simulink model "rocket_sim"  (R2023a)
settings: Solver=VariableStepAuto  StartTime=0.0  StopTime=480  RelTol=1e-3
undefined symbols (not defined in the file or in its folder): Earth, WGS84
libraries: simulink x55, slpidlib x10, aerolibconvert2 x7, matrix_library x4, aerolibasang x3, aerolibtransform2 x2, aerolibatmos2 x2, shared6dof x1, sharedtransform x1
(part 2 of 3)

== system rocket_sim/制导模块/Subsystem ==
  Clock2 : Clock
  Constant10 : Constant  Value=549000
  Constant11 : Constant  Value=150
  Constant12 : Constant  Value=486000
  Constant13 : Constant  Value=405000
  Gain2 : Gain  Gain=2700
  Gain3 : Gain  Gain=900
  Sum4 : Sum  Inputs=|+-
  Sum5 : Sum  Inputs=|+-
  Sum6 : Sum  Inputs=|++
  Switch4 : Switch  Criteria=u2 > Threshold  Threshold=150  SaturateOnIntegerOverflow=off  InputSameDT=off
  Switch5 : Switch  Criteria=u2 > Threshold  Threshold=240  SaturateOnIntegerOverflow=off  InputSameDT=off
  Out1 : Outport
  wires:
  Sum6/1 -> Switch5/3
  Gain2/1 -> Switch4/3
  Clock2/1 -> Switch5/2, Sum5/1, Switch4/2, Gain2/1
  Sum5/1 -> Gain3/1
  Constant10/1 -> Sum4/1
  Gain3/1 -> Sum6/1
  Constant12/1 -> Switch5/1
  Switch5/1 -> Switch4/1
  Sum4/1 -> Out1/1
  Constant13/1 -> Sum6/2
  Switch4/1 -> Sum4/2
  Constant11/1 -> Sum5/2

== system rocket_sim/制导模块/Subsystem1 ==
  Clock1 : Clock
  Constant : Constant  Value=[7000000;0;0]
  Constant3 : Constant  Value=[0;0;0]
  Constant8 : Constant  Value=[2000000;0;0]
  Constant9 : Constant  Value=[800000;0;0]
  Switch1 : Switch  Threshold=315  SaturateOnIntegerOverflow=off  InputSameDT=off
  Switch2 : Switch  Threshold=150  SaturateOnIntegerOverflow=off  InputSameDT=off
  Switch3 : Switch  Threshold=240  SaturateOnIntegerOverflow=off  InputSameDT=off
  Out1 : Outport
  wires:
  Clock1/1 -> Switch1/2, Switch3/2, Switch2/2
  Switch1/1 -> Switch3/1
  Constant3/1 -> Switch1/3
  Constant8/1 -> Switch3/3
  Constant9/1 -> Switch1/1
  Constant/1 -> Switch2/3
  Switch3/1 -> Switch2/1
  Switch2/1 -> Out1/1

== system rocket_sim/动力系统模块/喷管 ==
  dm : Inport
  P0 : Inport  Port=2
  Pi : Inport  Port=3
  Fwg : Inport  Port=4
  Th : Inport  Port=5
  F01 : Subsystem
  S71 : Scope
  喷管 : MATLAB Function  TreatAsAtomicUnit=on
  F : Outport
  ve : Outport  Port=2
  wires:
  dm/1 -> 喷管/1(dm)
  喷管/1(F) -> F/1
  Pi/1 -> 喷管/3(Pi)
  P0/1 -> 喷管/2(P0)
  喷管/2(ve) -> ve/1
  Fwg/1 -> F01/1(Fwg)
  Th/1 -> F01/2(Th)
  F01/1(Fwg1) -> S71/1, 喷管/4(Fwg1)

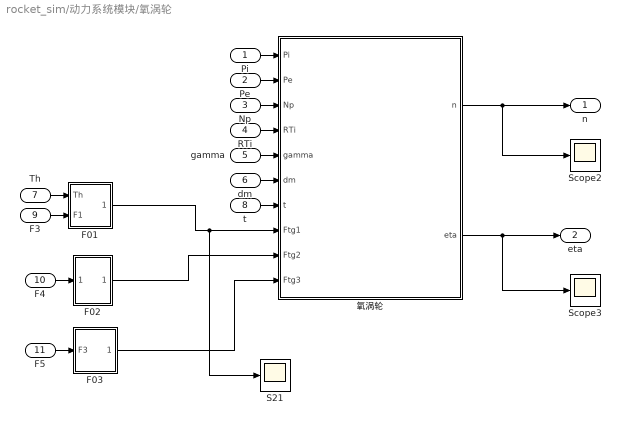
== system rocket_sim/动力系统模块/氧涡轮 ==
  Pi : Inport
  Pe : Inport  Port=2
  Np : Inport  Port=3
  RTi : Inport  Port=4
  gamma : Inport  Port=5
  dm : Inport  Port=6
  Th : Inport  Port=7
  t : Inport  Port=8
  F3 : Inport  Port=9
  F4 : Inport  Port=10
  F5 : Inport  Port=11
  F01 : Subsystem
  F02 : Subsystem
  F03 : Subsystem
  S21 : Scope
  Scope2 : Scope
  Scope3 : Scope
  氧涡轮 : MATLAB Function  TreatAsAtomicUnit=on
  n : Outport
  eta : Outport  Port=2
  wires:
  Pi/1 -> 氧涡轮/1(Pi)
  F03/1(Ftg3) -> 氧涡轮/10(Ftg3)
  Pe/1 -> 氧涡轮/2(Pe)
  Np/1 -> 氧涡轮/3(Np)
  F02/1(Ftg2) -> 氧涡轮/9(Ftg2)
  Th/1 -> F01/1(Th)
  t/1 -> 氧涡轮/7(t)
  F01/1(Ftg1) -> S21/1, 氧涡轮/8(Ftg1)
  F3/1 -> F01/2(F1)
  F4/1 -> F02/1(F2)
  RTi/1 -> 氧涡轮/4(RTi)
  F5/1 -> F03/1(F3)
  氧涡轮/2(eta) -> Scope3/1, eta/1
  dm/1 -> 氧涡轮/6(dm)
  氧涡轮/1(n) -> Scope2/1, n/1
  gamma/1 -> 氧涡轮/5(gamma)

== system rocket_sim/动力系统模块/液氧主阀 ==
  Pi : Inport
  dmi : Inport  Port=2
  Th : Inport  Port=3
  Constant : Constant
  F01 : Subsystem
  MATLAB Function : MATLAB Function  TreatAsAtomicUnit=on
  Memory : Memory
  S151 : Scope
  Pe : Outport
  dmo : Outport  Port=2
  wires:
  dmi/1 -> MATLAB Function/2(dmi)
  Pi/1 -> MATLAB Function/1(Pi)
  MATLAB Function/1(Pe) -> Pe/1
  Th/1 -> F01/1(Th)
  Constant/1 -> F01/2(Fv)
  F01/1(Fv1) -> S151/1, MATLAB Function/3(Fv1)
  Memory/1 -> dmo/1
  MATLAB Function/2(dmo) -> Memory/1

== system rocket_sim/动力系统模块/液氧泵 ==
  Pi : Inport
  n : Inport  Port=2
  Th : Inport  Port=3
  F1 : Inport  Port=4
  dm : Inport  Port=5
  F01 : Subsystem
  Memory : Memory
  S11 : Scope
  液氧泵 : MATLAB Function  TreatAsAtomicUnit=on
  Pe : Outport
  Np : Outport  Port=2
  dm02 : Outport  Port=3
  wires:
  Pi/1 -> 液氧泵/1(Pi)
  n/1 -> 液氧泵/3(n)
  F01/1(F) -> S11/1, 液氧泵/4(Fp1)
  液氧泵/1(Pe) -> Pe/1
  [dm] -> 液氧泵/2(dm)
  液氧泵/2(Np) -> Memory/1
  Memory/1 -> Np/1
  F1/1 -> F01/2(F1)
  Th/1 -> F01/1(Th)
  dm/1 -> [dm]
  [dm] -> dm02/1

== system rocket_sim/动力系统模块/液氧管路 ==
  P_i : Inport
  dm_i : Inport  Port=2
  Th : Inport  Port=3
  Constant6 : Constant
  F : Constant
  F01 : Subsystem
  Gain : Gain  Gain=0.02
  Integrator2 : Integrator
  MATLAB Function : MATLAB Function  TreatAsAtomicUnit=on
  Memory : Memory
  S141 : Scope
  dm_o : Outport
  P_e : Outport  Port=2
  dm_s1 : Outport  Port=3
  wires:
  P_i/1 -> MATLAB Function/1(P_i)
  Constant6/1 -> MATLAB Function/5(Fl2)
  MATLAB Function/2(P_e) -> P_e/1
  Integrator2/1 -> MATLAB Function/3(m)
  dm_i/1 -> Integrator2/1, MATLAB Function/2(dm_i)
  F01/1(F) -> S141/1, MATLAB Function/4(Fl1)
  Th/1 -> F01/1(Th)
  Gain/1 -> dm_s1/1
  MATLAB Function/1(dm_o) -> Memory/1
  Memory/1 -> Gain/1, dm_o/1
  F/1 -> F01/2(F1)

== system rocket_sim/动力系统模块/液氧贮箱 ==
  Band-Limited White Noise1 : simulink/Sources/Band-Limited White Noise  Cov=[0.1]  Ts=1  seed=[23341]
  Constant9 : Constant  Value=0.45
  Integrator1 : Integrator
  Step : Step  Time=0  After=214.06  SampleTime=0
  Sum : Sum  Inputs=|++
  σ1 : Gain  Gain=1e-3
  Po : Outport
  dm : Outport  Port=2
  wires:
  Constant9/1 -> Po/1
  Integrator1/1 -> σ1/1
  Band-Limited White Noise1/1 -> Integrator1/1
  Step/1 -> Sum/1
  Sum/1 -> dm/1
  σ1/1 -> Sum/2

== system rocket_sim/动力系统模块/煤油主阀 ==
  Pi : Inport
  dmi : Inport  Port=2
  Th : Inport  Port=3
  Fv : Inport  Port=4
  F01 : Subsystem
  MATLAB Function : MATLAB Function  TreatAsAtomicUnit=on
  Memory : Memory
  S41 : Scope
  Pe : Outport
  dmo : Outport  Port=2
  wires:
  F01/1(Fv1) -> S41/1, MATLAB Function/3(Fv1)
  dmi/1 -> MATLAB Function/2(dmi)
  Fv/1 -> F01/2(Fv)
  Pi/1 -> MATLAB Function/1(Pi)
  MATLAB Function/1(Pe) -> Pe/1
  Th/1 -> F01/1(Th)
  Memory/1 -> dmo/1
  MATLAB Function/2(dmo) -> Memory/1

== system rocket_sim/动力系统模块/煤油泵 ==
  Pi : Inport
  n : Inport  Port=2
  Th : Inport  Port=3
  dm : Inport  Port=4
  Constant : Constant
  F01 : Subsystem
  Memory : Memory
  S161 : Scope
  煤油泵 : MATLAB Function  TreatAsAtomicUnit=on
  Pe : Outport
  Np : Outport  Port=2
  dm12 : Outport  Port=3
  wires:
  Pi/1 -> 煤油泵/1(Pi)
  n/1 -> 煤油泵/3(n)
  F01/1(F) -> S161/1, 煤油泵/4(Fp1)
  煤油泵/1(Pe) -> Pe/1
  [dm] -> 煤油泵/2(dm)
  煤油泵/2(Np) -> Memory/1
  Memory/1 -> Np/1
  Constant/1 -> F01/2(F1)
  Th/1 -> F01/1(Th)
  dm/1 -> [dm]
  [dm] -> dm12/1

== system rocket_sim/动力系统模块/煤油涡轮 ==
  Pi : Inport
  Pe : Inport  Port=2
  Np : Inport  Port=3
  RTi : Inport  Port=4
  gamma : Inport  Port=5
  dm : Inport  Port=6
  Th : Inport  Port=7
  t : Inport  Port=8
  Constant : Constant
  Constant1 : Constant
  Constant2 : Constant
  F01 : Subsystem
  F02 : Subsystem
  F03 : Subsystem
  S171 : Scope
  Scope2 : Scope
  Scope3 : Scope
  氧涡轮 : MATLAB Function  TreatAsAtomicUnit=on
  n : Outport
  eta : Outport  Port=2
  wires:
  Pi/1 -> 氧涡轮/1(Pi)
  F03/1(Ftg3) -> 氧涡轮/10(Ftg3)
  Pe/1 -> 氧涡轮/2(Pe)
  Np/1 -> 氧涡轮/3(Np)
  F02/1(Ftg2) -> 氧涡轮/9(Ftg2)
  Th/1 -> F01/1(Th)
  t/1 -> 氧涡轮/7(t)
  F01/1(Ftg1) -> S171/1, 氧涡轮/8(Ftg1)
  RTi/1 -> 氧涡轮/4(RTi)
  氧涡轮/2(eta) -> Scope3/1, eta/1
  dm/1 -> 氧涡轮/6(dm)
  氧涡轮/1(n) -> Scope2/1, n/1
  gamma/1 -> 氧涡轮/5(gamma)
  Constant/1 -> F01/2(F1)
  Constant1/1 -> F02/1(F2)
  Constant2/1 -> F03/1(F3)

== system rocket_sim/动力系统模块/煤油管路 ==
  P_i : Inport
  dm_i : Inport  Port=2
  Th : Inport  Port=3
  Fl1 : Inport  Port=4
  Constant6 : Constant
  F01 : Subsystem
  Gain : Gain  Gain=0.02
  Integrator2 : Integrator
  MATLAB Function : MATLAB Function  TreatAsAtomicUnit=on
  Memory : Memory
  S31 : Scope
  dm_o : Outport
  P_e : Outport  Port=2
  dm_s1 : Outport  Port=3
  wires:
  P_i/1 -> MATLAB Function/1(P_i)
  Constant6/1 -> MATLAB Function/5(Fl2)
  MATLAB Function/2(P_e) -> P_e/1
  Integrator2/1 -> MATLAB Function/3(m)
  dm_i/1 -> Integrator2/1, MATLAB Function/2(dm_i)
  F01/1(F) -> S31/1, MATLAB Function/4(Fl1)
  Th/1 -> F01/1(Th)
  Fl1/1 -> F01/2(F1)
  Gain/1 -> dm_s1/1
  MATLAB Function/1(dm_o) -> Memory/1
  Memory/1 -> Gain/1, dm_o/1

== system rocket_sim/动力系统模块/煤油贮箱 ==
  Band-Limited White Noise1 : simulink/Sources/Band-Limited White Noise  Cov=[0.1]  Ts=1  seed=[23341]
  Constant9 : Constant  Value=0.31
  Integrator1 : Integrator
  Step : Step  Time=0  After=95.39  SampleTime=0
  Sum : Sum  Inputs=|++
  σ1 : Gain  Gain=1e-3
  Po : Outport
  dm : Outport  Port=2
  wires:
  Constant9/1 -> Po/1
  Band-Limited White Noise1/1 -> Integrator1/1
  Integrator1/1 -> σ1/1
  Step/1 -> Sum/1
  σ1/1 -> Sum/2
  Sum/1 -> dm/1

== system rocket_sim/动力系统模块/燃气发生器 ==
  dmo : Inport
  dmf : Inport  Port=2
  dmg : Inport  Port=3
  Pe : Inport  Port=4
  Th : Inport  Port=5
  F5 : Inport  Port=6
  Constant : Constant
  F01 : Subsystem
  S51 : Scope
  Scope : Scope
  燃气发生器 : MATLAB Function  TreatAsAtomicUnit=on
  gamma : Outport
  RT : Outport  Port=2
  dme : Outport  Port=3
  P : Outport  Port=4
  wires:
  dmg/1 -> 燃气发生器/3(dmg)
  Pe/1 -> 燃气发生器/4(Pe)
  燃气发生器/4(P) -> P/1
  dmo/1 -> 燃气发生器/1(dmo)
  dmf/1 -> 燃气发生器/2(dmf)
  Constant/1 -> 燃气发生器/5(Fg1)
  燃气发生器/1(gamma) -> gamma/1
  燃气发生器/2(RT) -> RT/1
  燃气发生器/3(dme) -> dme/1
  Th/1 -> F01/1(Th)
  F5/1 -> F01/2(F5)
  F01/1(Fg2) -> S51/1, 燃气发生器/6(Fg2)

== system rocket_sim/动力系统模块/燃烧室 ==
  dmo : Inport
  dmf : Inport  Port=2
  dmg : Inport  Port=3
  Th : Inport  Port=4
  Fr : Inport  Port=5
  F01 : Subsystem
  S61 : Scope
  燃烧室 : MATLAB Function  TreatAsAtomicUnit=on
  Pe : Outport
  dm : Outport  Port=2
  wires:
  dmg/1 -> 燃烧室/3(dmg)
  dmf/1 -> 燃烧室/2(dmf)
  燃烧室/1(Pe) -> Pe/1
  燃烧室/2(dm) -> dm/1
  dmo/1 -> 燃烧室/1(dmo)
  F01/1(Fr1) -> S61/1, 燃烧室/4(Fr1)
  Th/1 -> F01/1(Th)
  Fr/1 -> F01/2(Fr)

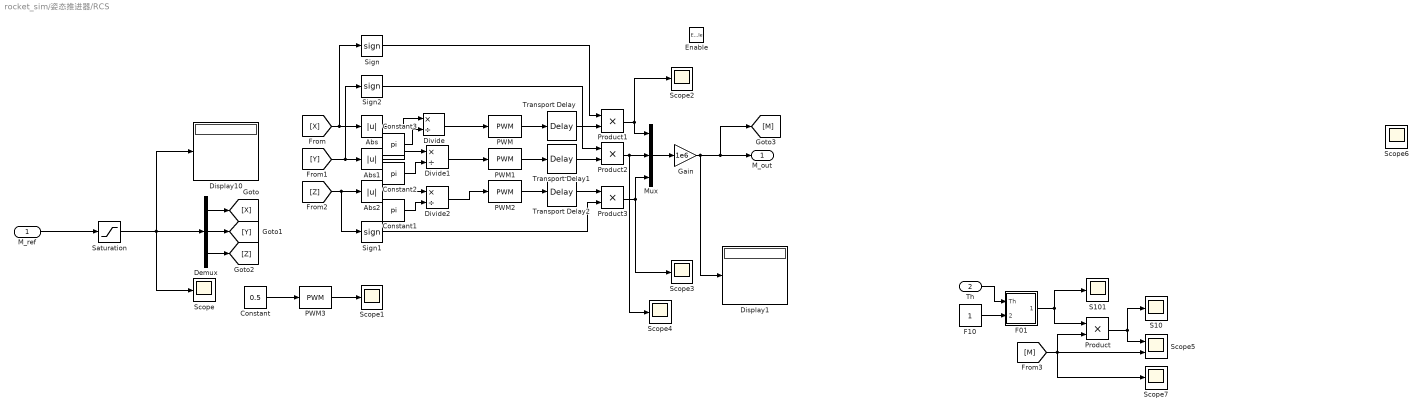
== system rocket_sim/姿态推进器/RCS ==
  M_ref : Inport
  Th : Inport  Port=2
  Enable : EnablePort
  Abs : Abs  SaturateOnIntegerOverflow=off
  Abs1 : Abs  SaturateOnIntegerOverflow=off
  Abs2 : Abs  SaturateOnIntegerOverflow=off
  Constant : Constant  Value=0.5
  Constant1 : Constant  Value=pi
  Constant2 : Constant  Value=pi
  Constant3 : Constant  Value=pi
  Demux : Demux  Outputs=3
  Display1 : Display
  Display10 : Display
  Divide : Product  Inputs=*/
  Divide1 : Product  Inputs=*/
  Divide2 : Product  Inputs=*/
  F01 : Subsystem
  F10 : Constant
  Gain : Gain  Gain=1e6
  Mux : Mux  Inputs=3
  PWM : simulink/Discontinuities/PWM  DisableCoverage=on  Period=1  InitialDelay=0  DisallowZeroDutyCycle=off  RunAtFixedTimeIntervals=off  SampleTime=0.1
  PWM1 : simulink/Discontinuities/PWM  DisableCoverage=on  Period=1  InitialDelay=0  DisallowZeroDutyCycle=off  RunAtFixedTimeIntervals=off  SampleTime=0.1
  PWM2 : simulink/Discontinuities/PWM  DisableCoverage=on  Period=1  InitialDelay=0  DisallowZeroDutyCycle=off  RunAtFixedTimeIntervals=off  SampleTime=0.1
  PWM3 : simulink/Discontinuities/PWM  DisableCoverage=on  Period=40  InitialDelay=0  DisallowZeroDutyCycle=off  RunAtFixedTimeIntervals=off  SampleTime=0.1
  Product{,1..3} (4 alike) : Product
  S10 : Scope
  S101 : Scope
  Saturation : Saturate  UpperLimit=3e10  LowerLimit=-3e10
  Scope{,1..4,6..7} (7 alike) : Scope
  Scope5 : Scope  NumInputPorts=2
  Sign : Signum
  Sign1 : Signum
  Sign2 : Signum
  Transport Delay : TransportDelay
  Transport Delay1 : TransportDelay
  Transport Delay2 : TransportDelay
  M_out : Outport
  wires:
  M_ref/1 -> Saturation/1
  Saturation/1 -> Demux/1, Display10/1, Scope/1
  PWM/1 -> Transport Delay/1
  PWM1/1 -> Transport Delay1/1
  PWM2/1 -> Transport Delay2/1
  Mux/1 -> Gain/1
  Gain/1 -> Display1/1, [M], M_out/1
  Constant/1 -> PWM3/1
  PWM3/1 -> Scope1/1
  Demux/1 -> [X]
  Demux/2 -> [Y]
  Demux/3 -> [Z]
  [X] -> Sign/1, Abs/1
  [Y] -> Sign2/1, Abs1/1
  [Z] -> Sign1/1, Abs2/1
  Transport Delay/1 -> Product1/2
  Sign/1 -> Product1/1
  Transport Delay1/1 -> Product2/2
  Sign2/1 -> Product2/1
  Transport Delay2/1 -> Product3/1
  Sign1/1 -> Product3/2
  Product1/1 -> Mux/1, Scope2/1
  Product2/1 -> Mux/2, Scope4/1
  Product3/1 -> Scope3/1, Mux/3
  Abs/1 -> Divide/1
  Divide/1 -> PWM/1
  Divide1/1 -> PWM1/1
  Abs1/1 -> Divide1/1
  Abs2/1 -> Divide2/1
  Divide2/1 -> PWM2/1
  Constant1/1 -> Divide2/2
  Constant2/1 -> Divide1/2
  Constant3/1 -> Divide/2
  [M] -> Scope7/1, Product/2, Scope5/2
  Product/1 -> Scope5/1, S10/1
  Th/1 -> F01/1(Th)
  F10/1 -> F01/2(In2)
  F01/1(Out1) -> Product/1, S101/1

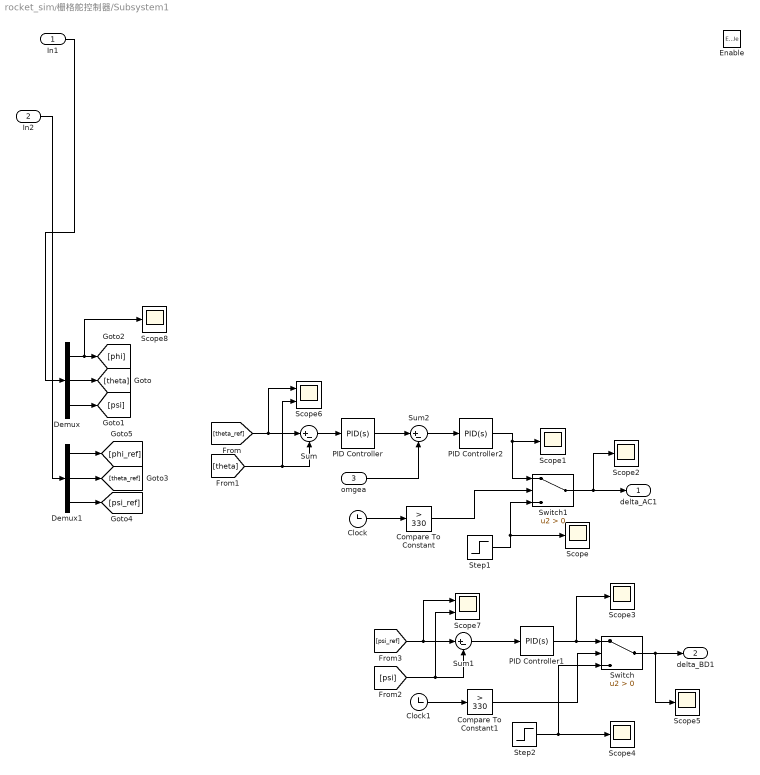
== system rocket_sim/栅格舵控制器/Subsystem1 ==
  In1 : Inport
  In2 : Inport  Port=2
  omgea : Inport  Port=3
  Enable : EnablePort
  Clock : Clock
  Clock1 : Clock
  Compare To Constant : simulink/Logic and Bit Operations/Compare To Constant  relop=>  const=330  OutDataTypeStr=boolean
  Compare To Constant1 : simulink/Logic and Bit Operations/Compare To Constant  relop=>  const=330  OutDataTypeStr=boolean
  Demux : Demux  Outputs=3
  Demux1 : Demux  Outputs=3
  PID Controller : slpidlib/PID Controller  Controller=PID  Form=Parallel  TimeDomain=Continuous-time  UseExternalTs=off  SampleTime=-1  IntegratorMethod=Forward Euler  FilterMethod=Forward Euler  ControllerParametersSource=internal  P=10  I=10  UseKiTs=off  D=10  N=100  UseFilter=on  TunerSelectOption=Transfer Function Based (PID Tuner App)  InitialConditionSource=internal  InitialConditionForIntegrator=0  InitialConditionForFilter=0  DifferentiatorICPrevScaledInput=0  ExternalReset=none  TrackingMode=off  Kt=1  LimitOutput=off  SatLimitsSource=internal  UpperSaturationLimit=inf  LowerSaturationLimit=-inf  LinearizeAsGain=on  AntiWindupMode=none  Kb=1  LimitIntegrator=off  UpperIntegratorSaturationLimit=inf  LowerIntegratorSaturationLimit=-inf  POutMin=[]  POutMax=[]  IOutMin=[]  IOutMax=[]  DOutMin=[]  DOutMax=[]  NOutMin=[]  NOutMax=[]  SumOutMin=[]  SumOutMax=[]  SaturationOutMin=[]  SaturationOutMax=[]  PParamMin=[]  PParamMax=[]  IParamMin=[]  IParamMax=[]  DParamMin=[]  DParamMax=[]  NParamMin=[]  NParamMax=[]  KbParamMin=[]  KbParamMax=[]  KtParamMin=[]  KtParamMax=[]  KbOutMin=[]  KbOutMax=[]  KtOutMin=[]  KtOutMax=[]  IntegratorOutMin=[]  IntegratorOutMax=[]  FilterOutMin=[]  FilterOutMax=[]  SumI1OutMin=[]  SumI1OutMax=[]  SumI2OutMin=[]  SumI2OutMax=[]  SumI3OutMin=[]  SumI3OutMax=[]  SumI4OutMin=[]  SumI4OutMax=[]  SumDOutMin=[]  SumDOutMax=[]  DifferentiatorOutMin=[]  DifferentiatorOutMax=[]  FilterDiffOutCoefMin=[]  FilterDiffOutCoefMax=[]  ReciprocalOutMin=[]  ReciprocalOutMax=[]  SumDenOutMin=[]  SumDenOutMax=[]  SumNumOutMin=[]  SumNumOutMax=[]  DivideOutMin=[]  DivideOutMax=[]  UdiffTsProdOutMin=[]  UdiffTsProdOutMax=[]  NTsProdOutMin=[]  NTsProdOutMax=[]  UintegralTsProdOutMin=[]  UintegralTsProdOutMax=[]  UngainTsProdOutMin=[]  UngainTsProdOutMax=[]  ClampingZeroOutDataTypeStr=Inherit: Inherit via back propagation  ClampingZeroOutMin=[]  ClampingZeroOutMax=[]  FilterDenConstantOutDataTypeStr=Inherit: Inherit via back propagation  FilterDenConstantOutMin=[]  FilterDenConstantOutMax=[]  PCopyOutDataTypeStr=Inherit: Inherit via back propagation  PCopyOutMin=[]  PCopyOutMax=[]  NCopyOutDataTypeStr=Inherit: Inherit via back propagation  NCopyOutMin=[]  NCopyOutMax=[]  IntegratorContinuousStateAttributes=''  IntegratorStateMustResolveToSignalObject=off  IntegratorRTWStateStorageClass=Auto  FilterContinuousStateAttributes=''  FilterStateMustResolveToSignalObject=off  FilterRTWStateStorageClass=Auto  ParallelPVariant=InternalParameters  IdealPVariant=Disabled  IVariant=InternalParameters  DVariant=InternalParameters  IntegratorVariant=Continuous  SatVariant=Disabled  AWVariant=Passthrough  PCopyVariant=Disabled  TRVariant=Disabled  FdbkBlocksVariant=Forward  IdealPFdbkVariant=Disabled  SatFdbkVariant=Disabled  DerivativeFilterVariant=ContFilter  NVariant=InternalParameters  NCopyVariant=Disabled  FilterICVariant=InternalICsFilter  IntegratorICVariant=InternalICs  ExternalResetVariant=Disabled  TRSumVariant=Passthrough  SumFdbkVariant=Disabled  SumVariant=Sum_PID  TsampFilterVariant=InternalTs  TsampNgainVariant=Passthrough  TsampIntegralVariant=Disabled_SignalSpec  ExternalSaturationOutDataTypeStr=Inherit: Same as second input
  PID Controller1 : slpidlib/PID Controller  Controller=PID  Form=Parallel  TimeDomain=Continuous-time  UseExternalTs=off  SampleTime=-1  IntegratorMethod=Forward Euler  FilterMethod=Forward Euler  ControllerParametersSource=internal  P=0  I=0  UseKiTs=off  D=0  N=100  UseFilter=on  TunerSelectOption=Transfer Function Based (PID Tuner App)  InitialConditionSource=internal  InitialConditionForIntegrator=0  InitialConditionForFilter=0  DifferentiatorICPrevScaledInput=0  ExternalReset=none  TrackingMode=off  Kt=1  LimitOutput=off  SatLimitsSource=internal  UpperSaturationLimit=inf  LowerSaturationLimit=-inf  LinearizeAsGain=on  AntiWindupMode=none  Kb=1  LimitIntegrator=off  UpperIntegratorSaturationLimit=inf  LowerIntegratorSaturationLimit=-inf  POutMin=[]  POutMax=[]  IOutMin=[]  IOutMax=[]  DOutMin=[]  DOutMax=[]  NOutMin=[]  NOutMax=[]  SumOutMin=[]  SumOutMax=[]  SaturationOutMin=[]  SaturationOutMax=[]  PParamMin=[]  PParamMax=[]  IParamMin=[]  IParamMax=[]  DParamMin=[]  DParamMax=[]  NParamMin=[]  NParamMax=[]  KbParamMin=[]  KbParamMax=[]  KtParamMin=[]  KtParamMax=[]  KbOutMin=[]  KbOutMax=[]  KtOutMin=[]  KtOutMax=[]  IntegratorOutMin=[]  IntegratorOutMax=[]  FilterOutMin=[]  FilterOutMax=[]  SumI1OutMin=[]  SumI1OutMax=[]  SumI2OutMin=[]  SumI2OutMax=[]  SumI3OutMin=[]  SumI3OutMax=[]  SumI4OutMin=[]  SumI4OutMax=[]  SumDOutMin=[]  SumDOutMax=[]  DifferentiatorOutMin=[]  DifferentiatorOutMax=[]  FilterDiffOutCoefMin=[]  FilterDiffOutCoefMax=[]  ReciprocalOutMin=[]  ReciprocalOutMax=[]  SumDenOutMin=[]  SumDenOutMax=[]  SumNumOutMin=[]  SumNumOutMax=[]  DivideOutMin=[]  DivideOutMax=[]  UdiffTsProdOutMin=[]  UdiffTsProdOutMax=[]  NTsProdOutMin=[]  NTsProdOutMax=[]  UintegralTsProdOutMin=[]  UintegralTsProdOutMax=[]  UngainTsProdOutMin=[]  UngainTsProdOutMax=[]  ClampingZeroOutDataTypeStr=Inherit: Inherit via back propagation  ClampingZeroOutMin=[]  ClampingZeroOutMax=[]  FilterDenConstantOutDataTypeStr=Inherit: Inherit via back propagation  FilterDenConstantOutMin=[]  FilterDenConstantOutMax=[]  PCopyOutDataTypeStr=Inherit: Inherit via back propagation  PCopyOutMin=[]  PCopyOutMax=[]  NCopyOutDataTypeStr=Inherit: Inherit via back propagation  NCopyOutMin=[]  NCopyOutMax=[]  IntegratorContinuousStateAttributes=''  IntegratorStateMustResolveToSignalObject=off  IntegratorRTWStateStorageClass=Auto  FilterContinuousStateAttributes=''  FilterStateMustResolveToSignalObject=off  FilterRTWStateStorageClass=Auto  ParallelPVariant=InternalParameters  IdealPVariant=Disabled  IVariant=InternalParameters  DVariant=InternalParameters  IntegratorVariant=Continuous  SatVariant=Disabled  AWVariant=Passthrough  PCopyVariant=Disabled  TRVariant=Disabled  FdbkBlocksVariant=Forward  IdealPFdbkVariant=Disabled  SatFdbkVariant=Disabled  DerivativeFilterVariant=ContFilter  NVariant=InternalParameters  NCopyVariant=Disabled  FilterICVariant=InternalICsFilter  IntegratorICVariant=InternalICs  ExternalResetVariant=Disabled  TRSumVariant=Passthrough  SumFdbkVariant=Disabled  SumVariant=Sum_PID  TsampFilterVariant=InternalTs  TsampNgainVariant=Passthrough  TsampIntegralVariant=Disabled_SignalSpec  ExternalSaturationOutDataTypeStr=Inherit: Same as second input
  PID Controller2 : slpidlib/PID Controller  Controller=PID  Form=Parallel  TimeDomain=Continuous-time  UseExternalTs=off  SampleTime=-1  IntegratorMethod=Forward Euler  FilterMethod=Forward Euler  ControllerParametersSource=internal  P=1  I=0  UseKiTs=off  D=0  N=100  UseFilter=on  TunerSelectOption=Transfer Function Based (PID Tuner App)  InitialConditionSource=internal  InitialConditionForIntegrator=0  InitialConditionForFilter=0  DifferentiatorICPrevScaledInput=0  ExternalReset=none  TrackingMode=off  Kt=1  LimitOutput=off  SatLimitsSource=internal  UpperSaturationLimit=inf  LowerSaturationLimit=-inf  LinearizeAsGain=on  AntiWindupMode=none  Kb=1  LimitIntegrator=off  UpperIntegratorSaturationLimit=inf  LowerIntegratorSaturationLimit=-inf  POutMin=[]  POutMax=[]  IOutMin=[]  IOutMax=[]  DOutMin=[]  DOutMax=[]  NOutMin=[]  NOutMax=[]  SumOutMin=[]  SumOutMax=[]  SaturationOutMin=[]  SaturationOutMax=[]  PParamMin=[]  PParamMax=[]  IParamMin=[]  IParamMax=[]  DParamMin=[]  DParamMax=[]  NParamMin=[]  NParamMax=[]  KbParamMin=[]  KbParamMax=[]  KtParamMin=[]  KtParamMax=[]  KbOutMin=[]  KbOutMax=[]  KtOutMin=[]  KtOutMax=[]  IntegratorOutMin=[]  IntegratorOutMax=[]  FilterOutMin=[]  FilterOutMax=[]  SumI1OutMin=[]  SumI1OutMax=[]  SumI2OutMin=[]  SumI2OutMax=[]  SumI3OutMin=[]  SumI3OutMax=[]  SumI4OutMin=[]  SumI4OutMax=[]  SumDOutMin=[]  SumDOutMax=[]  DifferentiatorOutMin=[]  DifferentiatorOutMax=[]  FilterDiffOutCoefMin=[]  FilterDiffOutCoefMax=[]  ReciprocalOutMin=[]  ReciprocalOutMax=[]  SumDenOutMin=[]  SumDenOutMax=[]  SumNumOutMin=[]  SumNumOutMax=[]  DivideOutMin=[]  DivideOutMax=[]  UdiffTsProdOutMin=[]  UdiffTsProdOutMax=[]  NTsProdOutMin=[]  NTsProdOutMax=[]  UintegralTsProdOutMin=[]  UintegralTsProdOutMax=[]  UngainTsProdOutMin=[]  UngainTsProdOutMax=[]  ClampingZeroOutDataTypeStr=Inherit: Inherit via back propagation  ClampingZeroOutMin=[]  ClampingZeroOutMax=[]  FilterDenConstantOutDataTypeStr=Inherit: Inherit via back propagation  FilterDenConstantOutMin=[]  FilterDenConstantOutMax=[]  PCopyOutDataTypeStr=Inherit: Inherit via back propagation  PCopyOutMin=[]  PCopyOutMax=[]  NCopyOutDataTypeStr=Inherit: Inherit via back propagation  NCopyOutMin=[]  NCopyOutMax=[]  IntegratorContinuousStateAttributes=''  IntegratorStateMustResolveToSignalObject=off  IntegratorRTWStateStorageClass=Auto  FilterContinuousStateAttributes=''  FilterStateMustResolveToSignalObject=off  FilterRTWStateStorageClass=Auto  ParallelPVariant=InternalParameters  IdealPVariant=Disabled  IVariant=InternalParameters  DVariant=InternalParameters  IntegratorVariant=Continuous  SatVariant=Disabled  AWVariant=Passthrough  PCopyVariant=Disabled  TRVariant=Disabled  FdbkBlocksVariant=Forward  IdealPFdbkVariant=Disabled  SatFdbkVariant=Disabled  DerivativeFilterVariant=ContFilter  NVariant=InternalParameters  NCopyVariant=Disabled  FilterICVariant=InternalICsFilter  IntegratorICVariant=InternalICs  ExternalResetVariant=Disabled  TRSumVariant=Passthrough  SumFdbkVariant=Disabled  SumVariant=Sum_PID  TsampFilterVariant=InternalTs  TsampNgainVariant=Passthrough  TsampIntegralVariant=Disabled_SignalSpec  ExternalSaturationOutDataTypeStr=Inherit: Same as second input
  Scope{,1..5,8} (7 alike) : Scope
  Scope6 : Scope  NumInputPorts=2
  Scope7 : Scope  NumInputPorts=2
  Step1 : Step  Time=0  After=0  SampleTime=0
  Step2 : Step  Time=0  After=0  SampleTime=0
  Sum : Sum  Inputs=|+-
  Sum1 : Sum  Inputs=|+-
  Sum2 : Sum  Inputs=|+-
  Switch : Switch  Criteria=u2 > Threshold  SaturateOnIntegerOverflow=off  InputSameDT=off
  Switch1 : Switch  Criteria=u2 > Threshold  SaturateOnIntegerOverflow=off  InputSameDT=off
  delta_AC1 : Outport
  delta_BD1 : Outport  Port=2
  wires:
  Step1/1 -> Switch1/3, Scope/1
  Switch1/1 -> delta_AC1/1, Scope2/1
  Sum1/1 -> PID Controller1/1
  [theta_ref] -> Scope6/1, Sum/1
  Clock1/1 -> Compare To Constant1/1
  Switch/1 -> delta_BD1/1, Scope5/1
  PID Controller1/1 -> Scope3/1, Switch/1
  Demux/3 -> [psi]
  [theta] -> Scope6/2, Sum/2
  PID Controller2/1 -> Scope1/1, Switch1/1
  Demux1/2 -> [theta_ref]
  [psi] -> Scope7/2, Sum1/2
  Clock/1 -> Compare To Constant/1
  Compare To Constant/1 -> Switch1/2
  Demux1/3 -> [psi_ref]
  Sum2/1 -> PID Controller2/1
  Step2/1 -> Scope4/1, Switch/3
  Demux/2 -> [theta]
  In1/1 -> Demux/1
  [psi_ref] -> Scope7/1, Sum1/1
  Compare To Constant1/1 -> Switch/2
  PID Controller/1 -> Sum2/1
  Sum/1 -> PID Controller/1
  Demux/1 -> Scope8/1, [phi]
  omgea/1 -> Sum2/2
  Demux1/1 -> [phi_ref]
  In2/1 -> Demux1/1

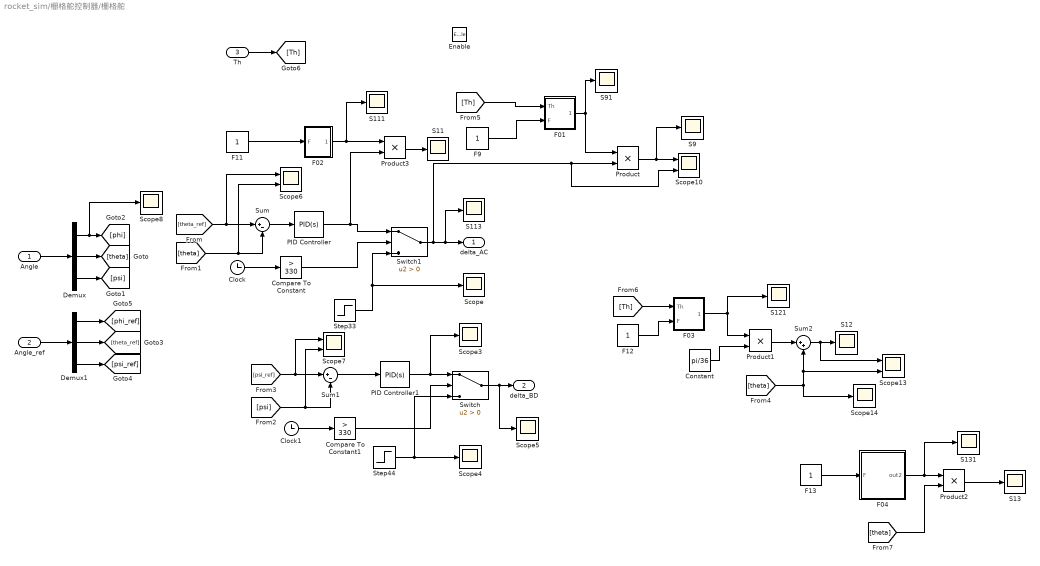
== system rocket_sim/栅格舵控制器/栅格舵 ==
  Angle : Inport
  Angle_ref : Inport  Port=2
  Th : Inport  Port=3
  Enable : EnablePort
  Clock : Clock
  Clock1 : Clock
  Compare To Constant : simulink/Logic and Bit Operations/Compare To Constant  relop=>  const=330  OutDataTypeStr=boolean
  Compare To Constant1 : simulink/Logic and Bit Operations/Compare To Constant  relop=>  const=330  OutDataTypeStr=boolean
  Constant : Constant  Value=pi/36
  Demux : Demux  Outputs=3
  Demux1 : Demux  Outputs=3
  F01 : Subsystem
  F02 : Subsystem
  F03 : Subsystem
  F04 : Subsystem
  F{9,11..13} (4 alike) : Constant
  PID Controller : slpidlib/PID Controller  Controller=PID  Form=Parallel  TimeDomain=Continuous-time  UseExternalTs=off  SampleTime=-1  IntegratorMethod=Forward Euler  FilterMethod=Forward Euler  ControllerParametersSource=internal  P=0.016  I=0  UseKiTs=off  D=15  N=100  UseFilter=on  TunerSelectOption=Transfer Function Based (PID Tuner App)  InitialConditionSource=internal  InitialConditionForIntegrator=0  InitialConditionForFilter=0  DifferentiatorICPrevScaledInput=0  ExternalReset=none  TrackingMode=off  Kt=1  LimitOutput=off  SatLimitsSource=internal  UpperSaturationLimit=inf  LowerSaturationLimit=-inf  LinearizeAsGain=on  AntiWindupMode=none  Kb=1  LimitIntegrator=off  UpperIntegratorSaturationLimit=inf  LowerIntegratorSaturationLimit=-inf  POutMin=[]  POutMax=[]  IOutMin=[]  IOutMax=[]  DOutMin=[]  DOutMax=[]  NOutMin=[]  NOutMax=[]  SumOutMin=[]  SumOutMax=[]  SaturationOutMin=[]  SaturationOutMax=[]  PParamMin=[]  PParamMax=[]  IParamMin=[]  IParamMax=[]  DParamMin=[]  DParamMax=[]  NParamMin=[]  NParamMax=[]  KbParamMin=[]  KbParamMax=[]  KtParamMin=[]  KtParamMax=[]  KbOutMin=[]  KbOutMax=[]  KtOutMin=[]  KtOutMax=[]  IntegratorOutMin=[]  IntegratorOutMax=[]  FilterOutMin=[]  FilterOutMax=[]  SumI1OutMin=[]  SumI1OutMax=[]  SumI2OutMin=[]  SumI2OutMax=[]  SumI3OutMin=[]  SumI3OutMax=[]  SumI4OutMin=[]  SumI4OutMax=[]  SumDOutMin=[]  SumDOutMax=[]  DifferentiatorOutMin=[]  DifferentiatorOutMax=[]  FilterDiffOutCoefMin=[]  FilterDiffOutCoefMax=[]  ReciprocalOutMin=[]  ReciprocalOutMax=[]  SumDenOutMin=[]  SumDenOutMax=[]  SumNumOutMin=[]  SumNumOutMax=[]  DivideOutMin=[]  DivideOutMax=[]  UdiffTsProdOutMin=[]  UdiffTsProdOutMax=[]  NTsProdOutMin=[]  NTsProdOutMax=[]  UintegralTsProdOutMin=[]  UintegralTsProdOutMax=[]  UngainTsProdOutMin=[]  UngainTsProdOutMax=[]  ClampingZeroOutDataTypeStr=Inherit: Inherit via back propagation  ClampingZeroOutMin=[]  ClampingZeroOutMax=[]  FilterDenConstantOutDataTypeStr=Inherit: Inherit via back propagation  FilterDenConstantOutMin=[]  FilterDenConstantOutMax=[]  PCopyOutDataTypeStr=Inherit: Inherit via back propagation  PCopyOutMin=[]  PCopyOutMax=[]  NCopyOutDataTypeStr=Inherit: Inherit via back propagation  NCopyOutMin=[]  NCopyOutMax=[]  IntegratorContinuousStateAttributes=''  IntegratorStateMustResolveToSignalObject=off  IntegratorRTWStateStorageClass=Auto  FilterContinuousStateAttributes=''  FilterStateMustResolveToSignalObject=off  FilterRTWStateStorageClass=Auto  ParallelPVariant=InternalParameters  IdealPVariant=Disabled  IVariant=InternalParameters  DVariant=InternalParameters  IntegratorVariant=Continuous  SatVariant=Disabled  AWVariant=Passthrough  PCopyVariant=Disabled  TRVariant=Disabled  FdbkBlocksVariant=Forward  IdealPFdbkVariant=Disabled  SatFdbkVariant=Disabled  DerivativeFilterVariant=ContFilter  NVariant=InternalParameters  NCopyVariant=Disabled  FilterICVariant=InternalICsFilter  IntegratorICVariant=InternalICs  ExternalResetVariant=Disabled  TRSumVariant=Passthrough  SumFdbkVariant=Disabled  SumVariant=Sum_PID  TsampFilterVariant=InternalTs  TsampNgainVariant=Passthrough  TsampIntegralVariant=Disabled_SignalSpec  ExternalSaturationOutDataTypeStr=Inherit: Same as second input
  PID Controller1 : slpidlib/PID Controller  Controller=PID  Form=Parallel  TimeDomain=Continuous-time  UseExternalTs=off  SampleTime=-1  IntegratorMethod=Forward Euler  FilterMethod=Forward Euler  ControllerParametersSource=internal  P=0  I=0  UseKiTs=off  D=0  N=100  UseFilter=on  TunerSelectOption=Transfer Function Based (PID Tuner App)  InitialConditionSource=internal  InitialConditionForIntegrator=0  InitialConditionForFilter=0  DifferentiatorICPrevScaledInput=0  ExternalReset=none  TrackingMode=off  Kt=1  LimitOutput=off  SatLimitsSource=internal  UpperSaturationLimit=inf  LowerSaturationLimit=-inf  LinearizeAsGain=on  AntiWindupMode=none  Kb=1  LimitIntegrator=off  UpperIntegratorSaturationLimit=inf  LowerIntegratorSaturationLimit=-inf  POutMin=[]  POutMax=[]  IOutMin=[]  IOutMax=[]  DOutMin=[]  DOutMax=[]  NOutMin=[]  NOutMax=[]  SumOutMin=[]  SumOutMax=[]  SaturationOutMin=[]  SaturationOutMax=[]  PParamMin=[]  PParamMax=[]  IParamMin=[]  IParamMax=[]  DParamMin=[]  DParamMax=[]  NParamMin=[]  NParamMax=[]  KbParamMin=[]  KbParamMax=[]  KtParamMin=[]  KtParamMax=[]  KbOutMin=[]  KbOutMax=[]  KtOutMin=[]  KtOutMax=[]  IntegratorOutMin=[]  IntegratorOutMax=[]  FilterOutMin=[]  FilterOutMax=[]  SumI1OutMin=[]  SumI1OutMax=[]  SumI2OutMin=[]  SumI2OutMax=[]  SumI3OutMin=[]  SumI3OutMax=[]  SumI4OutMin=[]  SumI4OutMax=[]  SumDOutMin=[]  SumDOutMax=[]  DifferentiatorOutMin=[]  DifferentiatorOutMax=[]  FilterDiffOutCoefMin=[]  FilterDiffOutCoefMax=[]  ReciprocalOutMin=[]  ReciprocalOutMax=[]  SumDenOutMin=[]  SumDenOutMax=[]  SumNumOutMin=[]  SumNumOutMax=[]  DivideOutMin=[]  DivideOutMax=[]  UdiffTsProdOutMin=[]  UdiffTsProdOutMax=[]  NTsProdOutMin=[]  NTsProdOutMax=[]  UintegralTsProdOutMin=[]  UintegralTsProdOutMax=[]  UngainTsProdOutMin=[]  UngainTsProdOutMax=[]  ClampingZeroOutDataTypeStr=Inherit: Inherit via back propagation  ClampingZeroOutMin=[]  ClampingZeroOutMax=[]  FilterDenConstantOutDataTypeStr=Inherit: Inherit via back propagation  FilterDenConstantOutMin=[]  FilterDenConstantOutMax=[]  PCopyOutDataTypeStr=Inherit: Inherit via back propagation  PCopyOutMin=[]  PCopyOutMax=[]  NCopyOutDataTypeStr=Inherit: Inherit via back propagation  NCopyOutMin=[]  NCopyOutMax=[]  IntegratorContinuousStateAttributes=''  IntegratorStateMustResolveToSignalObject=off  IntegratorRTWStateStorageClass=Auto  FilterContinuousStateAttributes=''  FilterStateMustResolveToSignalObject=off  FilterRTWStateStorageClass=Auto  ParallelPVariant=InternalParameters  IdealPVariant=Disabled  IVariant=InternalParameters  DVariant=InternalParameters  IntegratorVariant=Continuous  SatVariant=Disabled  AWVariant=Passthrough  PCopyVariant=Disabled  TRVariant=Disabled  FdbkBlocksVariant=Forward  IdealPFdbkVariant=Disabled  SatFdbkVariant=Disabled  DerivativeFilterVariant=ContFilter  NVariant=InternalParameters  NCopyVariant=Disabled  FilterICVariant=InternalICsFilter  IntegratorICVariant=InternalICs  ExternalResetVariant=Disabled  TRSumVariant=Passthrough  SumFdbkVariant=Disabled  SumVariant=Sum_PID  TsampFilterVariant=InternalTs  TsampNgainVariant=Passthrough  TsampIntegralVariant=Disabled_SignalSpec  ExternalSaturationOutDataTypeStr=Inherit: Same as second input
  Product{,1..3} (4 alike) : Product
  S{9,11..13,91,111,113,121,131} (9 alike) : Scope
  Scope{,3..5,8,14} (6 alike) : Scope
  Scope{6..7,10,13} (4 alike) : Scope  NumInputPorts=2
  Step33 : Step  Time=0  After=0  SampleTime=0
  Step44 : Step  Time=0  After=0  SampleTime=0
  Sum : Sum  Inputs=|+-
  Sum1 : Sum  Inputs=|+-
  Sum2 : Sum  Inputs=|++
  Switch : Switch  Criteria=u2 > Threshold  SaturateOnIntegerOverflow=off  InputSameDT=off
  Switch1 : Switch  Criteria=u2 > Threshold  SaturateOnIntegerOverflow=off  InputSameDT=off
  delta_AC : Outport
  delta_BD : Outport  Port=2
  wires:
  Demux1/2 -> [theta_ref]
  Angle_ref/1 -> Demux1/1
  Demux1/3 -> [psi_ref]
  Angle/1 -> Demux/1
  Demux/3 -> [psi]
  Demux/2 -> [theta]
  [theta_ref] -> Scope6/1, Sum/1
  [theta] -> Scope6/2, Sum/2
  Demux/1 -> Scope8/1, [phi]
  [psi_ref] -> Scope7/1, Sum1/1
  [psi] -> Scope7/2, Sum1/2
  Demux1/1 -> [phi_ref]
  Clock/1 -> Compare To Constant/1
  Switch1/1 -> Scope10/2, Product/2, S113/1, delta_AC/1
  Step33/1 -> Switch1/3, Scope/1
  Sum/1 -> PID Controller/1
  Sum1/1 -> PID Controller1/1
  PID Controller1/1 -> Scope3/1, Switch/1
  Clock1/1 -> Compare To Constant1/1
  Compare To Constant1/1 -> Switch/2
  Step44/1 -> Scope4/1, Switch/3
  Switch/1 -> Scope5/1, delta_BD/1
  Compare To Constant/1 -> Switch1/2
  F01/1(Out1) -> Product/1, S91/1
  F9/1 -> F01/2(F)
  Product/1 -> S9/1, Scope10/1
  Th/1 -> [Th]
  [Th] -> F01/1(Th)
  [Th] -> F03/1(Th)
  F03/1(Out1) -> S121/1, Product1/1
  [theta] -> Scope14/1, Sum2/2, Scope13/2
  F12/1 -> F03/2(F)
  Product1/1 -> Sum2/1
  Sum2/1 -> Scope13/1, S12/1
  Constant/1 -> Product1/2
  F04/1(out2) -> S131/1, Product2/1
  [theta] -> Product2/2
  Product2/1 -> S13/1
  F13/1 -> F04/1(F)
  F11/1 -> F02/1(F)
  F02/1(out2) -> S111/1, Product3/1
  PID Controller/1 -> Product3/2, Switch1/1
  Product3/1 -> S11/1

== system rocket_sim/TVC模块/F01/故障 ==
  Th : Inport
  Band-Limited White Noise : simulink/Sources/Band-Limited White Noise  Cov=[0.1]  Ts=0.1  seed=[23341]
  Clock1 : Clock
  Constant : Constant  Value=0.8
  Gain3 : Gain  Gain=-4e-05
  Gain4 : Gain  Gain=0.001
  Integrator : Integrator
  Scope : Scope
  Sum : Sum  Inputs=|+++
  Sum1 : Sum  Inputs=|++
  Out1 : Outport
  wires:
  Sum/1 -> Scope/1, Out1/1
  Sum1/1 -> Gain3/1
  Th/1 -> Sum1/2
  Gain3/1 -> Sum/1
  Band-Limited White Noise/1 -> Integrator/1
  Integrator/1 -> Gain4/1
  Clock1/1 -> Sum1/1
  Gain4/1 -> Sum/2
  Constant/1 -> Sum/3

== system rocket_sim/TVC模块/F01/退化 ==
  Th : Inport
  Band-Limited White Noise : simulink/Sources/Band-Limited White Noise  Cov=[0.1]  Ts=0.1  seed=[23341]
  Clock1 : Clock
  Constant : Constant
  Gain3 : Gain  Gain=-4e-05
  Gain4 : Gain  Gain=0.001
  Integrator : Integrator
  Sum : Sum  Inputs=|+++
  Sum1 : Sum  Inputs=|++
  Out1 : Outport
  wires:
  Sum/1 -> Out1/1
  Sum1/1 -> Gain3/1
  Th/1 -> Sum1/2
  Gain3/1 -> Sum/1
  Band-Limited White Noise/1 -> Integrator/1
  Integrator/1 -> Gain4/1
  Clock1/1 -> Sum1/1
  Gain4/1 -> Sum/2
  Constant/1 -> Sum/3

== system rocket_sim/TVC模块/Subsystem/故障 ==
  Th1 : Inport
  Band-Limited White Noise : simulink/Sources/Band-Limited White Noise  Cov=[0.1]  Ts=0.1  seed=[23341]
  Clock : Clock
  Constant : Constant
  Constant5 : Constant  Value=2
  Gain : Gain  Gain=-1.2153e-04
  Gain3 : Gain  Gain=0.0001
  Integrator : Integrator
  Product3 : Product
  Sum : Sum  Inputs=|+++
  Sum1 : Sum  Inputs=|++
  Out1 : Outport
  wires:
  Product3/1 -> Out1/1
  Sum1/1 -> Gain/1
  Gain3/1 -> Sum/2
  Constant5/1 -> Product3/1
  Integrator/1 -> Gain3/1
  Clock/1 -> Sum1/1
  Sum/1 -> Product3/2
  Band-Limited White Noise/1 -> Integrator/1
  Th1/1 -> Sum1/2
  Constant/1 -> Sum/3
  Gain/1 -> Sum/1

== system rocket_sim/TVC模块/Subsystem/退化 ==
  Th : Inport
  Band-Limited White Noise : simulink/Sources/Band-Limited White Noise  Cov=[0.1]  Ts=0.1  seed=[23341]
  Clock : Clock
  Constant : Constant
  Constant4 : Constant  Value=16
  Gain : Gain  Gain=-1.2153e-04
  Gain3 : Gain  Gain=0.001
  Integrator : Integrator
  Product3 : Product
  Scope : Scope
  Sum : Sum  Inputs=|+++
  Sum1 : Sum  Inputs=|++
  Out1 : Outport
  wires:
  Clock/1 -> Sum1/1
  Band-Limited White Noise/1 -> Integrator/1
  Gain3/1 -> Sum/2
  Constant4/1 -> Product3/1
  Th/1 -> Sum1/2
  Integrator/1 -> Gain3/1
  Sum/1 -> Scope/1, Product3/2
  Product3/1 -> Out1/1
  Sum1/1 -> Gain/1
  Gain/1 -> Sum/1
  Constant/1 -> Sum/3

== system rocket_sim/冷气推进器控制器/Subsystem1/故障 ==
  Th1 : Inport
  Band-Limited White Noise : simulink/Sources/Band-Limited White Noise  Cov=[0.1]  Ts=0.1  seed=[23341]
  Clock : Clock
  Constant : Constant
  Constant5 : Constant  Value=2
  Gain : Gain  Gain=-1.2153e-04
  Gain3 : Gain  Gain=0.0001
  Integrator : Integrator
  Product3 : Product
  Sum : Sum  Inputs=|+++
  Sum1 : Sum  Inputs=|++
  Out1 : Outport
  wires:
  Product3/1 -> Out1/1
  Sum1/1 -> Gain/1
  Gain3/1 -> Sum/2
  Constant5/1 -> Product3/1
  Integrator/1 -> Gain3/1
  Clock/1 -> Sum1/1
  Sum/1 -> Product3/2
  Band-Limited White Noise/1 -> Integrator/1
  Th1/1 -> Sum1/2
  Constant/1 -> Sum/3
  Gain/1 -> Sum/1

== system rocket_sim/冷气推进器控制器/Subsystem1/退化 ==
  Th : Inport
  Band-Limited White Noise : simulink/Sources/Band-Limited White Noise  Cov=[0.1]  Ts=0.1  seed=[23341]
  Clock : Clock
  Constant : Constant
  Constant4 : Constant  Value=16
  Gain : Gain  Gain=-1.2153e-04
  Gain3 : Gain  Gain=0.001
  Integrator : Integrator
  Product3 : Product
  Scope : Scope
  Sum : Sum  Inputs=|+++
  Sum1 : Sum  Inputs=|++
  Out1 : Outport
  wires:
  Clock/1 -> Sum1/1
  Band-Limited White Noise/1 -> Integrator/1
  Gain3/1 -> Sum/2
  Constant4/1 -> Product3/1
  Th/1 -> Sum1/2
  Integrator/1 -> Gain3/1
  Sum/1 -> Scope/1, Product3/2
  Product3/1 -> Out1/1
  Sum1/1 -> Gain/1
  Gain/1 -> Sum/1
  Constant/1 -> Sum/3

== system rocket_sim/动力系统模块/喷管/F01 ==
  Fwg : Inport
  Th : Inport  Port=2
  Constant : Constant  Value=0
  Scope : Scope
  Step1 : Step  Time=200  SampleTime=0
  Step2 : Step  Time=300  SampleTime=0
  Switch : Switch  Criteria=u2 > Threshold  SaturateOnIntegerOverflow=off  InputSameDT=off
  Switch1 : Switch  Criteria=u2 > Threshold  SaturateOnIntegerOverflow=off  InputSameDT=off
  Switch2 : Switch  Criteria=u2 > Threshold  SaturateOnIntegerOverflow=off  InputSameDT=off
  故障 : Subsystem
  退化 : Subsystem
  Fwg1 : Outport
  wires:
  Switch2/1 -> Switch1/2
  Step1/1 -> Switch2/3
  故障/1(Out1) -> Switch1/1
  Constant/1 -> Switch2/1
  Th/1 -> 故障/1(Th), 退化/1(Th)
  Switch1/1 -> Switch/3
  Fwg/1 -> Switch2/2
  Step2/1 -> Switch/2
  退化/1(Out1) -> Switch1/3, Scope/1, Switch/1
  Switch/1 -> Fwg1/1

== system rocket_sim/动力系统模块/氧涡轮/F01 ==
  Th : Inport
  F1 : Inport  Port=2
  Constant2 : Constant  Value=0
  Step1 : Step  Time=200  SampleTime=0
  Step2 : Step  Time=300  SampleTime=0
  Switch : Switch  Criteria=u2 > Threshold  SaturateOnIntegerOverflow=off  InputSameDT=off
  Switch1 : Switch  Criteria=u2 > Threshold  SaturateOnIntegerOverflow=off  InputSameDT=off
  Switch2 : Switch  Criteria=u2 > Threshold  SaturateOnIntegerOverflow=off  InputSameDT=off
  故障 : Subsystem
  退化 : Subsystem
  Ftg1 : Outport
  wires:
  退化/1(Out1) -> Switch1/3, Switch/1
  Switch1/1 -> Switch/3
  Step2/1 -> Switch/2
  Constant2/1 -> Switch2/1
  Step1/1 -> Switch2/3
  Th/1 -> 故障/1(Th), 退化/1(Th)
  Switch2/1 -> Switch1/2
  故障/1(Out1) -> Switch1/1
  Switch/1 -> Ftg1/1
  F1/1 -> Switch2/2

== system rocket_sim/动力系统模块/氧涡轮/F02 ==
  F2 : Inport
  Constant1 : Constant  Value=0
  Constant2 : Constant  Value=0.2
  Constant4 : Constant  Value=0
  Step1 : Step  Time=100  SampleTime=0
  Step2 : Step  Time=200  SampleTime=0
  Switch : Switch  Criteria=u2 > Threshold  SaturateOnIntegerOverflow=off  InputSameDT=off
  Switch1 : Switch  Criteria=u2 > Threshold  SaturateOnIntegerOverflow=off  InputSameDT=off
  Switch2 : Switch  Criteria=u2 > Threshold  SaturateOnIntegerOverflow=off  InputSameDT=off
  Ftg2 : Outport
  wires:
  Step2/1 -> Switch/2
  Constant4/1 -> Switch2/1
  Constant1/1 -> Switch1/3, Switch/1
  F2/1 -> Switch2/2
  Switch2/1 -> Switch1/2
  Constant2/1 -> Switch1/1
  Step1/1 -> Switch2/3
  Switch1/1 -> Switch/3
  Switch/1 -> Ftg2/1

== system rocket_sim/动力系统模块/氧涡轮/F03 ==
  F3 : Inport
  Constant2 : Constant
  Constant4 : Constant  Value=0.8
  Constant6 : Constant  Value=0
  Step1 : Step  Time=100  SampleTime=0
  Step2 : Step  Time=200  SampleTime=0
  Switch : Switch  Criteria=u2 > Threshold  SaturateOnIntegerOverflow=off  InputSameDT=off
  Switch1 : Switch  Criteria=u2 > Threshold  SaturateOnIntegerOverflow=off  InputSameDT=off
  Switch2 : Switch  Criteria=u2 > Threshold  SaturateOnIntegerOverflow=off  InputSameDT=off
  Ftg3 : Outport
  wires:
  F3/1 -> Switch2/2
  Constant2/1 -> Switch1/3, Switch/1
  Switch2/1 -> Switch1/2
  Constant6/1 -> Switch2/1
  Switch1/1 -> Switch/3
  Step2/1 -> Switch/2
  Switch/1 -> Ftg3/1
  Constant4/1 -> Switch1/1
  Step1/1 -> Switch2/3

== system rocket_sim/动力系统模块/液氧主阀/F01 ==
  Th : Inport
  Fv : Inport  Port=2
  Constant : Constant  Value=0
  Step1 : Step  Time=200  SampleTime=0
  Step2 : Step  Time=300  SampleTime=0
  Switch : Switch  Criteria=u2 > Threshold  SaturateOnIntegerOverflow=off  InputSameDT=off
  Switch1 : Switch  Criteria=u2 > Threshold  SaturateOnIntegerOverflow=off  InputSameDT=off
  Switch2 : Switch  Criteria=u2 > Threshold  SaturateOnIntegerOverflow=off  InputSameDT=off
  故障 : Subsystem
  退化 : Subsystem
  Fv1 : Outport
  wires:
  Switch1/1 -> Switch/3
  退化/1(Out1) -> Switch1/3, Switch/1
  Th/1 -> 故障/1(Th), 退化/1(Th)
  故障/1(Out1) -> Switch1/1
  Switch/1 -> Fv1/1
  Step2/1 -> Switch/2
  Switch2/1 -> Switch1/2
  Step1/1 -> Switch2/3
  Constant/1 -> Switch2/1
  Fv/1 -> Switch2/2

== system rocket_sim/动力系统模块/液氧泵/F01 ==
  Th : Inport
  F1 : Inport  Port=2
  Constant : Constant  Value=0
  Saturation : Saturate  UpperLimit=1  LowerLimit=0.5
  Scope : Scope
  Step1 : Step  Time=100  SampleTime=0
  Step2 : Step  Time=480  SampleTime=0
  Switch : Switch  Criteria=u2 > Threshold  SaturateOnIntegerOverflow=off  InputSameDT=off
  Switch1 : Switch  Criteria=u2 > Threshold  SaturateOnIntegerOverflow=off  InputSameDT=off
  Switch2 : Switch  Criteria=u2 > Threshold  SaturateOnIntegerOverflow=off  InputSameDT=off
  故障 : Subsystem
  退化 : Subsystem
  F : Outport
  wires:
  Switch/1 -> Saturation/1
  Saturation/1 -> F/1, Scope/1
  退化/1(Out1) -> Switch1/3, Switch/1
  Switch1/1 -> Switch/3
  Step2/1 -> Switch/2
  Th/1 -> 故障/1(Th), 退化/1(Th)
  故障/1(Out1) -> Switch1/1
  Switch2/1 -> Switch1/2
  Step1/1 -> Switch2/3
  F1/1 -> Switch2/2
  Constant/1 -> Switch2/1

== system rocket_sim/动力系统模块/液氧管路/F01 ==
  Th : Inport
  F1 : Inport  Port=2
  Constant : Constant  Value=0
  Saturation : Saturate  UpperLimit=1  LowerLimit=0.5
  Scope : Scope
  Scope1 : Scope
  Step1 : Step  Time=200  SampleTime=0
  Step2 : Step  Time=300  SampleTime=0
  Switch : Switch  Criteria=u2 > Threshold  SaturateOnIntegerOverflow=off  InputSameDT=off
  Switch1 : Switch  Criteria=u2 > Threshold  SaturateOnIntegerOverflow=off  InputSameDT=off
  Switch2 : Switch  Criteria=u2 > Threshold  SaturateOnIntegerOverflow=off  InputSameDT=off
  故障 : Subsystem
  退化 : Subsystem
  F : Outport
  wires:
  Switch/1 -> Saturation/1
  Saturation/1 -> Scope/1, F/1
  退化/1(Out1) -> Switch1/3, Scope1/1, Switch/1
  Switch1/1 -> Switch/3
  Step2/1 -> Switch/2
  Th/1 -> 故障/1(Th), 退化/1(Th)
  故障/1(Out1) -> Switch1/1
  Switch2/1 -> Switch1/2
  Step1/1 -> Switch2/3
  F1/1 -> Switch2/2
  Constant/1 -> Switch2/1

== system rocket_sim/动力系统模块/煤油主阀/F01 ==
  Th : Inport
  Fv : Inport  Port=2
  Constant : Constant  Value=0
  Step1 : Step  Time=200  SampleTime=0
  Step2 : Step  Time=300  SampleTime=0
  Switch : Switch  Criteria=u2 > Threshold  SaturateOnIntegerOverflow=off  InputSameDT=off
  Switch1 : Switch  Criteria=u2 > Threshold  SaturateOnIntegerOverflow=off  InputSameDT=off
  Switch2 : Switch  Criteria=u2 > Threshold  SaturateOnIntegerOverflow=off  InputSameDT=off
  故障 : Subsystem
  退化 : Subsystem
  Fv1 : Outport
  wires:
  Switch1/1 -> Switch/3
  退化/1(Out1) -> Switch1/3, Switch/1
  Th/1 -> 故障/1(Th), 退化/1(Th)
  故障/1(Out1) -> Switch1/1
  Switch/1 -> Fv1/1
  Step2/1 -> Switch/2
  Switch2/1 -> Switch1/2
  Step1/1 -> Switch2/3
  Constant/1 -> Switch2/1
  Fv/1 -> Switch2/2

== system rocket_sim/动力系统模块/煤油泵/F01 ==
  Th : Inport
  F1 : Inport  Port=2
  Constant : Constant  Value=0
  Saturation : Saturate  UpperLimit=1  LowerLimit=0.5
  Scope : Scope
  Step1 : Step  Time=200  SampleTime=0
  Step2 : Step  Time=300  SampleTime=0
  Switch : Switch  Criteria=u2 > Threshold  SaturateOnIntegerOverflow=off  InputSameDT=off
  Switch1 : Switch  Criteria=u2 > Threshold  SaturateOnIntegerOverflow=off  InputSameDT=off
  Switch2 : Switch  Criteria=u2 > Threshold  SaturateOnIntegerOverflow=off  InputSameDT=off
  故障 : Subsystem
  退化 : Subsystem
  F : Outport
  wires:
  Switch/1 -> Saturation/1
  Saturation/1 -> Scope/1, F/1
  退化/1(Out1) -> Switch1/3, Switch/1
  Switch1/1 -> Switch/3
  Step2/1 -> Switch/2
  Th/1 -> 故障/1(Th), 退化/1(Th)
  故障/1(Out1) -> Switch1/1
  Switch2/1 -> Switch1/2
  Step1/1 -> Switch2/3
  F1/1 -> Switch2/2
  Constant/1 -> Switch2/1

== system rocket_sim/动力系统模块/煤油涡轮/F01 ==
  Th : Inport
  F1 : Inport  Port=2
  Constant2 : Constant  Value=0
  Step1 : Step  Time=200  SampleTime=0
  Step2 : Step  Time=300  SampleTime=0
  Switch : Switch  Criteria=u2 > Threshold  SaturateOnIntegerOverflow=off  InputSameDT=off
  Switch1 : Switch  Criteria=u2 > Threshold  SaturateOnIntegerOverflow=off  InputSameDT=off
  Switch2 : Switch  Criteria=u2 > Threshold  SaturateOnIntegerOverflow=off  InputSameDT=off
  故障 : Subsystem
  退化 : Subsystem
  Ftg1 : Outport
  wires:
  退化/1(Out1) -> Switch1/3, Switch/1
  Switch1/1 -> Switch/3
  Step2/1 -> Switch/2
  Constant2/1 -> Switch2/1
  Step1/1 -> Switch2/3
  Th/1 -> 故障/1(Th), 退化/1(Th)
  Switch2/1 -> Switch1/2
  故障/1(Out1) -> Switch1/1
  Switch/1 -> Ftg1/1
  F1/1 -> Switch2/2

== system rocket_sim/动力系统模块/煤油涡轮/F02 ==
  F2 : Inport
  Constant1 : Constant  Value=0
  Constant2 : Constant  Value=0.2
  Constant4 : Constant  Value=0
  Step1 : Step  Time=100  SampleTime=0
  Step2 : Step  Time=200  SampleTime=0
  Switch : Switch  Criteria=u2 > Threshold  SaturateOnIntegerOverflow=off  InputSameDT=off
  Switch1 : Switch  Criteria=u2 > Threshold  SaturateOnIntegerOverflow=off  InputSameDT=off
  Switch2 : Switch  Criteria=u2 > Threshold  SaturateOnIntegerOverflow=off  InputSameDT=off
  Ftg2 : Outport
  wires:
  Step2/1 -> Switch/2
  Constant4/1 -> Switch2/1
  Constant1/1 -> Switch1/3, Switch/1
  F2/1 -> Switch2/2
  Switch2/1 -> Switch1/2
  Constant2/1 -> Switch1/1
  Step1/1 -> Switch2/3
  Switch1/1 -> Switch/3
  Switch/1 -> Ftg2/1

== system rocket_sim/动力系统模块/煤油涡轮/F03 ==
  F3 : Inport
  Constant2 : Constant
  Constant4 : Constant  Value=0.8
  Constant6 : Constant  Value=0
  Step1 : Step  Time=100  SampleTime=0
  Step2 : Step  Time=200  SampleTime=0
  Switch : Switch  Criteria=u2 > Threshold  SaturateOnIntegerOverflow=off  InputSameDT=off
  Switch1 : Switch  Criteria=u2 > Threshold  SaturateOnIntegerOverflow=off  InputSameDT=off
  Switch2 : Switch  Criteria=u2 > Threshold  SaturateOnIntegerOverflow=off  InputSameDT=off
  Ftg3 : Outport
  wires:
  F3/1 -> Switch2/2
  Constant2/1 -> Switch1/3, Switch/1
  Switch2/1 -> Switch1/2
  Constant6/1 -> Switch2/1
  Switch1/1 -> Switch/3
  Step2/1 -> Switch/2
  Switch/1 -> Ftg3/1
  Constant4/1 -> Switch1/1
  Step1/1 -> Switch2/3

== system rocket_sim/动力系统模块/煤油管路/F01 ==
  Th : Inport
  F1 : Inport  Port=2
  Constant : Constant  Value=0
  Saturation : Saturate  UpperLimit=1  LowerLimit=0.5
  Scope : Scope
  Step1 : Step  Time=200  SampleTime=0
  Step2 : Step  Time=300  SampleTime=0
  Switch : Switch  Criteria=u2 > Threshold  SaturateOnIntegerOverflow=off  InputSameDT=off
  Switch1 : Switch  Criteria=u2 > Threshold  SaturateOnIntegerOverflow=off  InputSameDT=off
  Switch2 : Switch  Criteria=u2 > Threshold  SaturateOnIntegerOverflow=off  InputSameDT=off
  故障 : Subsystem
  退化 : Subsystem
  F : Outport
  wires:
  Switch/1 -> Saturation/1
  Saturation/1 -> Scope/1, F/1
  退化/1(Out1) -> Switch1/3, Switch/1
  Switch1/1 -> Switch/3
  Step2/1 -> Switch/2
  Th/1 -> 故障/1(Th), 退化/1(Th)
  故障/1(Out1) -> Switch1/1
  Switch2/1 -> Switch1/2
  Step1/1 -> Switch2/3
  F1/1 -> Switch2/2
  Constant/1 -> Switch2/1

== system rocket_sim/动力系统模块/燃气发生器/F01 ==
  Th : Inport
  F5 : Inport  Port=2
  Constant1 : Constant  Value=0
  Scope : Scope
  Step1 : Step  Time=200  SampleTime=0
  Step2 : Step  Time=480  SampleTime=0
  Switch : Switch  Criteria=u2 > Threshold  SaturateOnIntegerOverflow=off  InputSameDT=off
  Switch1 : Switch  Criteria=u2 > Threshold  SaturateOnIntegerOverflow=off  InputSameDT=off
  Switch2 : Switch  Criteria=u2 > Threshold  SaturateOnIntegerOverflow=off  InputSameDT=off
  故障 : Subsystem
  退化 : Subsystem
  Fg2 : Outport
  wires:
  Switch2/1 -> Switch1/2
  F5/1 -> Switch2/2
  退化/1(Fg2) -> Switch1/3, Scope/1, Switch/1
  Th/1 -> 故障/1(Th), 退化/1(Th)
  Step2/1 -> Switch/2
  Step1/1 -> Switch2/3
  故障/1(Fg2) -> Switch1/1
  Constant1/1 -> Switch2/1
  Switch1/1 -> Switch/3
  Switch/1 -> Fg2/1

== system rocket_sim/动力系统模块/燃烧室/F01 ==
  Th : Inport
  Fr : Inport  Port=2
  Constant : Constant  Value=0
  Step1 : Step  Time=200  SampleTime=0
  Step2 : Step  Time=300  SampleTime=0
  Switch : Switch  Criteria=u2 > Threshold  SaturateOnIntegerOverflow=off  InputSameDT=off
  Switch1 : Switch  Criteria=u2 > Threshold  SaturateOnIntegerOverflow=off  InputSameDT=off
  Switch2 : Switch  Criteria=u2 > Threshold  SaturateOnIntegerOverflow=off  InputSameDT=off
  故障 : Subsystem
  退化 : Subsystem
  Fr1 : Outport
  wires:
  Step2/1 -> Switch/2
  退化/1(Out1) -> Switch1/3, Switch/1
  Step1/1 -> Switch2/3
  Th/1 -> 故障/1(Th), 退化/1(Th)
  Switch2/1 -> Switch1/2
  故障/1(Out1) -> Switch1/1
  Fr/1 -> Switch2/2
  Switch1/1 -> Switch/3
  Constant/1 -> Switch2/1
  Switch/1 -> Fr1/1

== system rocket_sim/姿态推进器/RCS/F01 ==
  Th : Inport
  In2 : Inport  Port=2
  Constant4 : Constant  Value=0
  Step1 : Step  Time=100  SampleTime=0
  Step2 : Step  Time=200  SampleTime=0
  Switch : Switch  Criteria=u2 > Threshold  SaturateOnIntegerOverflow=off  InputSameDT=off
  Switch1 : Switch  Criteria=u2 > Threshold  SaturateOnIntegerOverflow=off  InputSameDT=off
  Switch2 : Switch  Criteria=u2 > Threshold  SaturateOnIntegerOverflow=off  InputSameDT=off
  故障 : Subsystem
  退化 : Subsystem
  Out1 : Outport
  wires:
  退化/1(Out1) -> Switch1/3, Switch/1
  Step1/1 -> Switch2/3
  Step2/1 -> Switch/2
  故障/1(Out1) -> Switch1/1
  Switch1/1 -> Switch/3
  Th/1 -> 故障/1(Th), 退化/1(Th)
  Constant4/1 -> Switch2/1
  Switch2/1 -> Switch1/2
  In2/1 -> Switch2/2
  Switch/1 -> Out1/1
